simulink model "DroneModelSimulink"  (R2024b)
settings: Solver=VariableStepAuto  StartTime=0.0  StopTime=10  RelTol=1e-3
libraries: slpidlib x3, simulink x1
settings Model: Creator=ewert  LastModifiedBy=asus
settings SolverCC: AlgebraicLoopSolver=TrustRegion
settings DataIOCC: ReturnWorkspaceOutputs=off
settings DebuggingCC: UnconnectedInputMsg=warning  UnconnectedOutputMsg=warning  UnconnectedLineMsg=warning  ArithmeticOperatorsInVariantConditions=warning
settings ModelReferenceCC: EnableRefExpFcnMdlSchedulingChecks=on
settings SFSimCC: SimUseLocalCustomCode=off  CustomCodeUndefinedFunction=UseInterfaceOnly
settings RTWCC: RTWUseLocalCustomCode=off  GPUComputeCapability=3.5
settings CodeAppCC: StateflowObjectComments=on

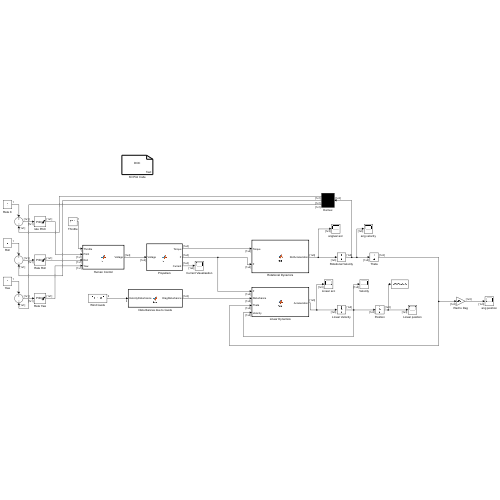
[thumbnail: Simulink's stored preview of the top-level diagram]
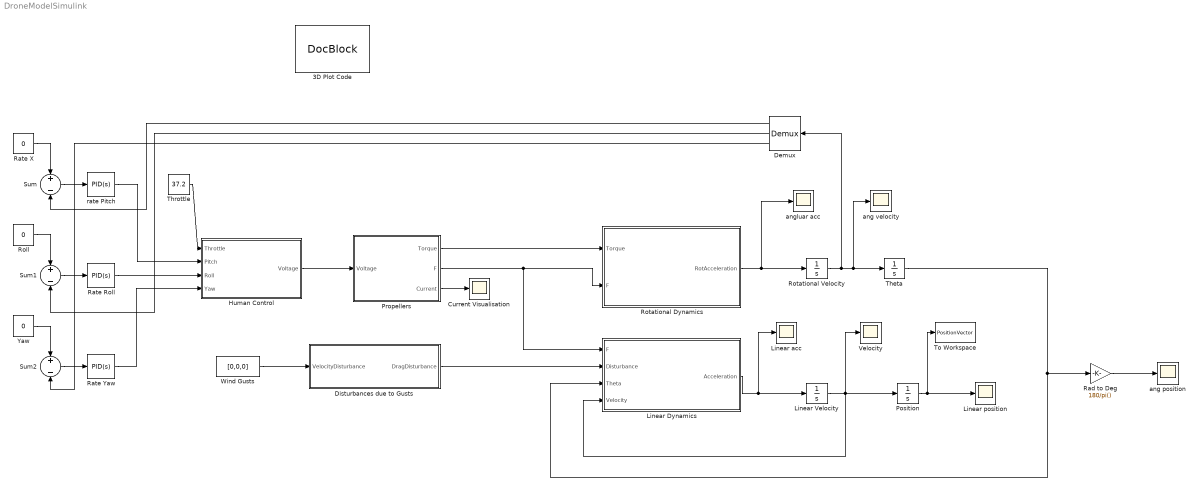
== system DroneModelSimulink ==
  3D Plot Code : simulink/Model-Wide Utilities/DocBlock  DocumentType=Text
      content=|
      | % Use this sample code once the simulation is completed to export 3D plot and visualize the drone's behavior
      | %----------------------------------
      | data3D = squeeze(PositionVector);
      | X = data3D(1, :);
      | Y = data3D(2, :);
      | Z = data3D(3, :);
      | figure;
      | plot3(X, Y, Z, '-r');
      | grid on;
      | xlabel('X');
      | ylabel('Y');
      | zlabel('Z');
      | title('3D Plot from Pos Data');
      | %----------------------------------
  "Current Visualisation " : Scope
  Demux : Demux  Outputs=3
  Disturbances due to Gusts : MATLAB Function  TreatAsAtomicUnit=on
  Human Control : MATLAB Function  TreatAsAtomicUnit=on
  Linear Dynamics : MATLAB Function  TreatAsAtomicUnit=on
  Linear Velocity : Integrator
  Linear acc : Scope
  Linear position : Scope
  Position : Integrator
  Propellers : MATLAB Function  TreatAsAtomicUnit=on
  Rad to Deg : Gain  Gain=180/pi()
  Rate Roll : slpidlib/PID Controller  Controller=PID  Form=Parallel  TimeDomain=Continuous-time  UseExternalTs=off  SampleTime=-1  IntegratorMethod=Forward Euler  FilterMethod=Forward Euler  ControllerParametersSource=internal  P=10  I=5  UseKiTs=off  D=0  UseExternalDerivativeSource=off  N=100  UseFilter=on  TunerSelectOption=Transfer Function Based (PID Tuner App)  InitialConditionSource=internal  InitialConditionForIntegrator=0  InitialConditionForFilter=0  DifferentiatorICPrevScaledInput=0  ExternalReset=none  TrackingMode=off  Kt=1  LimitOutput=on  SatLimitsSource=internal  UpperSaturationLimit=100  LowerSaturationLimit=0  LinearizeAsGain=on  AntiWindupMode=clamping  Kb=1  LimitIntegrator=off  UpperIntegratorSaturationLimit=inf  LowerIntegratorSaturationLimit=-inf  POutMin=[]  POutMax=[]  IOutMin=[]  IOutMax=[]  DOutMin=[]  DOutMax=[]  NOutMin=[]  NOutMax=[]  SumOutMin=[]  SumOutMax=[]  SaturationOutMin=[]  SaturationOutMax=[]  PParamMin=[]  PParamMax=[]  IParamMin=[]  IParamMax=[]  DParamMin=[]  DParamMax=[]  NParamMin=[]  NParamMax=[]  KbParamMin=[]  KbParamMax=[]  KtParamMin=[]  KtParamMax=[]  KbOutMin=[]  KbOutMax=[]  KtOutMin=[]  KtOutMax=[]  IntegratorOutMin=[]  IntegratorOutMax=[]  FilterOutMin=[]  FilterOutMax=[]  SumI1OutMin=[]  SumI1OutMax=[]  SumI2OutMin=[]  SumI2OutMax=[]  SumI3OutMin=[]  SumI3OutMax=[]  SumI4OutMin=[]  SumI4OutMax=[]  SumDOutMin=[]  SumDOutMax=[]  DifferentiatorOutMin=[]  DifferentiatorOutMax=[]  FilterDiffOutCoefMin=[]  FilterDiffOutCoefMax=[]  ReciprocalOutMin=[]  ReciprocalOutMax=[]  SumDenOutMin=[]  SumDenOutMax=[]  SumNumOutMin=[]  SumNumOutMax=[]  DivideOutMin=[]  DivideOutMax=[]  UdiffTsProdOutMin=[]  UdiffTsProdOutMax=[]  NTsProdOutMin=[]  NTsProdOutMax=[]  UintegralTsProdOutMin=[]  UintegralTsProdOutMax=[]  UngainTsProdOutMin=[]  UngainTsProdOutMax=[]  ClampingZeroOutDataTypeStr=Inherit: Inherit via back propagation  ClampingZeroOutMin=[]  ClampingZeroOutMax=[]  FilterDenConstantOutDataTypeStr=Inherit: Inherit via back propagation  FilterDenConstantOutMin=[]  FilterDenConstantOutMax=[]  PCopyOutDataTypeStr=Inherit: Inherit via back propagation  PCopyOutMin=[]  PCopyOutMax=[]  NCopyOutDataTypeStr=Inherit: Inherit via back propagation  NCopyOutMin=[]  NCopyOutMax=[]  IntegratorContinuousStateAttributes=''  IntegratorStateMustResolveToSignalObject=off  IntegratorRTWStateStorageClass=Auto  FilterContinuousStateAttributes=''  FilterStateMustResolveToSignalObject=off  FilterRTWStateStorageClass=Auto  ParallelPVariant=InternalParameters  IdealPVariant=Disabled  IVariant=InternalParameters  DVariant=InternalParameters  IntegratorVariant=Continuous  SatVariant=Enabled  AWVariant=ContClampingParallel  PCopyVariant=Disabled  TRVariant=Disabled  FdbkBlocksVariant=Forward  IdealPFdbkVariant=Disabled  SatFdbkVariant=Disabled  DerivativeFilterVariant=ContFilter  NVariant=InternalParameters  NCopyVariant=Disabled  FilterICVariant=InternalICsFilter  IntegratorICVariant=InternalICs  ExternalResetVariant=Disabled  TRSumVariant=Passthrough  SumFdbkVariant=Disabled  SumVariant=Sum_PID  TsampFilterVariant=InternalTs  TsampNgainVariant=Passthrough  TsampIntegralVariant=Disabled_SignalSpec  ExternalSaturationOutDataTypeStr=Inherit: Same as second input  DerivativeSourceVariant=ErrorSignal  PreIntVariant=InternalPreInt
  Rate X : Constant  Value=0
  Rate Yaw : slpidlib/PID Controller  Controller=PID  Form=Parallel  TimeDomain=Continuous-time  UseExternalTs=off  SampleTime=-1  IntegratorMethod=Forward Euler  FilterMethod=Forward Euler  ControllerParametersSource=internal  P=5  I=0.5  UseKiTs=off  D=0  UseExternalDerivativeSource=off  N=100  UseFilter=on  TunerSelectOption=Transfer Function Based (PID Tuner App)  InitialConditionSource=internal  InitialConditionForIntegrator=0  InitialConditionForFilter=0  DifferentiatorICPrevScaledInput=0  ExternalReset=none  TrackingMode=off  Kt=1  LimitOutput=on  SatLimitsSource=internal  UpperSaturationLimit=100  LowerSaturationLimit=0  LinearizeAsGain=on  AntiWindupMode=clamping  Kb=1  LimitIntegrator=off  UpperIntegratorSaturationLimit=inf  LowerIntegratorSaturationLimit=-inf  POutMin=[]  POutMax=[]  IOutMin=[]  IOutMax=[]  DOutMin=[]  DOutMax=[]  NOutMin=[]  NOutMax=[]  SumOutMin=[]  SumOutMax=[]  SaturationOutMin=[]  SaturationOutMax=[]  PParamMin=[]  PParamMax=[]  IParamMin=[]  IParamMax=[]  DParamMin=[]  DParamMax=[]  NParamMin=[]  NParamMax=[]  KbParamMin=[]  KbParamMax=[]  KtParamMin=[]  KtParamMax=[]  KbOutMin=[]  KbOutMax=[]  KtOutMin=[]  KtOutMax=[]  IntegratorOutMin=[]  IntegratorOutMax=[]  FilterOutMin=[]  FilterOutMax=[]  SumI1OutMin=[]  SumI1OutMax=[]  SumI2OutMin=[]  SumI2OutMax=[]  SumI3OutMin=[]  SumI3OutMax=[]  SumI4OutMin=[]  SumI4OutMax=[]  SumDOutMin=[]  SumDOutMax=[]  DifferentiatorOutMin=[]  DifferentiatorOutMax=[]  FilterDiffOutCoefMin=[]  FilterDiffOutCoefMax=[]  ReciprocalOutMin=[]  ReciprocalOutMax=[]  SumDenOutMin=[]  SumDenOutMax=[]  SumNumOutMin=[]  SumNumOutMax=[]  DivideOutMin=[]  DivideOutMax=[]  UdiffTsProdOutMin=[]  UdiffTsProdOutMax=[]  NTsProdOutMin=[]  NTsProdOutMax=[]  UintegralTsProdOutMin=[]  UintegralTsProdOutMax=[]  UngainTsProdOutMin=[]  UngainTsProdOutMax=[]  ClampingZeroOutDataTypeStr=Inherit: Inherit via back propagation  ClampingZeroOutMin=[]  ClampingZeroOutMax=[]  FilterDenConstantOutDataTypeStr=Inherit: Inherit via back propagation  FilterDenConstantOutMin=[]  FilterDenConstantOutMax=[]  PCopyOutDataTypeStr=Inherit: Inherit via back propagation  PCopyOutMin=[]  PCopyOutMax=[]  NCopyOutDataTypeStr=Inherit: Inherit via back propagation  NCopyOutMin=[]  NCopyOutMax=[]  IntegratorContinuousStateAttributes=''  IntegratorStateMustResolveToSignalObject=off  IntegratorRTWStateStorageClass=Auto  FilterContinuousStateAttributes=''  FilterStateMustResolveToSignalObject=off  FilterRTWStateStorageClass=Auto  ParallelPVariant=InternalParameters  IdealPVariant=Disabled  IVariant=InternalParameters  DVariant=InternalParameters  IntegratorVariant=Continuous  SatVariant=Enabled  AWVariant=ContClampingParallel  PCopyVariant=Disabled  TRVariant=Disabled  FdbkBlocksVariant=Forward  IdealPFdbkVariant=Disabled  SatFdbkVariant=Disabled  DerivativeFilterVariant=ContFilter  NVariant=InternalParameters  NCopyVariant=Disabled  FilterICVariant=InternalICsFilter  IntegratorICVariant=InternalICs  ExternalResetVariant=Disabled  TRSumVariant=Passthrough  SumFdbkVariant=Disabled  SumVariant=Sum_PID  TsampFilterVariant=InternalTs  TsampNgainVariant=Passthrough  TsampIntegralVariant=Disabled_SignalSpec  ExternalSaturationOutDataTypeStr=Inherit: Same as second input  DerivativeSourceVariant=ErrorSignal  PreIntVariant=InternalPreInt
  Roll : Constant  Value=0
  Rotational Dynamics : MATLAB Function  TreatAsAtomicUnit=on
  Rotational Velocity : Integrator
  Sum : Sum  Inputs=+-
  Sum1 : Sum  Inputs=+-
  Sum2 : Sum  Inputs=+-
  Theta : Integrator
  Throttle : Constant  Value=37.2
  To Workspace : ToWorkspace  VariableName=PositionVector  SampleTime=-1
      settings: Save2DSignal=2-D array (concatenate along first dimension)
  "Velocity " : Scope
  Wind Gusts : Constant  Value=[0,0,0]
  Yaw : Constant  Value=0
  ang position : Scope
  ang velocity : Scope
  angluar acc : Scope
  rate Pitch : slpidlib/PID Controller  Controller=PID  Form=Parallel  TimeDomain=Continuous-time  UseExternalTs=off  SampleTime=-1  IntegratorMethod=Forward Euler  FilterMethod=Forward Euler  ControllerParametersSource=internal  P=10  I=5  UseKiTs=off  D=0  UseExternalDerivativeSource=off  N=100  UseFilter=on  TunerSelectOption=Transfer Function Based (PID Tuner App)  InitialConditionSource=internal  InitialConditionForIntegrator=0  InitialConditionForFilter=0  DifferentiatorICPrevScaledInput=0  ExternalReset=none  TrackingMode=off  Kt=1  LimitOutput=on  SatLimitsSource=internal  UpperSaturationLimit=100  LowerSaturationLimit=0  LinearizeAsGain=on  AntiWindupMode=clamping  Kb=1  LimitIntegrator=off  UpperIntegratorSaturationLimit=inf  LowerIntegratorSaturationLimit=-inf  POutMin=[]  POutMax=[]  IOutMin=[]  IOutMax=[]  DOutMin=[]  DOutMax=[]  NOutMin=[]  NOutMax=[]  SumOutMin=[]  SumOutMax=[]  SaturationOutMin=[]  SaturationOutMax=[]  PParamMin=[]  PParamMax=[]  IParamMin=[]  IParamMax=[]  DParamMin=[]  DParamMax=[]  NParamMin=[]  NParamMax=[]  KbParamMin=[]  KbParamMax=[]  KtParamMin=[]  KtParamMax=[]  KbOutMin=[]  KbOutMax=[]  KtOutMin=[]  KtOutMax=[]  IntegratorOutMin=[]  IntegratorOutMax=[]  FilterOutMin=[]  FilterOutMax=[]  SumI1OutMin=[]  SumI1OutMax=[]  SumI2OutMin=[]  SumI2OutMax=[]  SumI3OutMin=[]  SumI3OutMax=[]  SumI4OutMin=[]  SumI4OutMax=[]  SumDOutMin=[]  SumDOutMax=[]  DifferentiatorOutMin=[]  DifferentiatorOutMax=[]  FilterDiffOutCoefMin=[]  FilterDiffOutCoefMax=[]  ReciprocalOutMin=[]  ReciprocalOutMax=[]  SumDenOutMin=[]  SumDenOutMax=[]  SumNumOutMin=[]  SumNumOutMax=[]  DivideOutMin=[]  DivideOutMax=[]  UdiffTsProdOutMin=[]  UdiffTsProdOutMax=[]  NTsProdOutMin=[]  NTsProdOutMax=[]  UintegralTsProdOutMin=[]  UintegralTsProdOutMax=[]  UngainTsProdOutMin=[]  UngainTsProdOutMax=[]  ClampingZeroOutDataTypeStr=Inherit: Inherit via back propagation  ClampingZeroOutMin=[]  ClampingZeroOutMax=[]  FilterDenConstantOutDataTypeStr=Inherit: Inherit via back propagation  FilterDenConstantOutMin=[]  FilterDenConstantOutMax=[]  PCopyOutDataTypeStr=Inherit: Inherit via back propagation  PCopyOutMin=[]  PCopyOutMax=[]  NCopyOutDataTypeStr=Inherit: Inherit via back propagation  NCopyOutMin=[]  NCopyOutMax=[]  IntegratorContinuousStateAttributes=''  IntegratorStateMustResolveToSignalObject=off  IntegratorRTWStateStorageClass=Auto  FilterContinuousStateAttributes=''  FilterStateMustResolveToSignalObject=off  FilterRTWStateStorageClass=Auto  ParallelPVariant=InternalParameters  IdealPVariant=Disabled  IVariant=InternalParameters  DVariant=InternalParameters  IntegratorVariant=Continuous  SatVariant=Enabled  AWVariant=ContClampingParallel  PCopyVariant=Disabled  TRVariant=Disabled  FdbkBlocksVariant=Forward  IdealPFdbkVariant=Disabled  SatFdbkVariant=Disabled  DerivativeFilterVariant=ContFilter  NVariant=InternalParameters  NCopyVariant=Disabled  FilterICVariant=InternalICsFilter  IntegratorICVariant=InternalICs  ExternalResetVariant=Disabled  TRSumVariant=Passthrough  SumFdbkVariant=Disabled  SumVariant=Sum_PID  TsampFilterVariant=InternalTs  TsampNgainVariant=Passthrough  TsampIntegralVariant=Disabled_SignalSpec  ExternalSaturationOutDataTypeStr=Inherit: Same as second input  DerivativeSourceVariant=ErrorSignal  PreIntVariant=InternalPreInt
  wires:
  Propellers/1(Torque) -> Rotational Dynamics/1(Torque)
  Propellers/2(F) -> Linear Dynamics/1(F), Rotational Dynamics/2(F)
  Rotational Dynamics/1(RotAcceleration) -> angluar acc/1, Rotational Velocity/1
  Rotational Velocity/1 -> Demux/1, ang velocity/1, Theta/1
  Theta/1 -> Rad to Deg/1, Linear Dynamics/3(Theta)
  Linear Dynamics/1(Acceleration) -> Linear acc/1, Linear Velocity/1
  Linear Velocity/1 -> "Velocity "/1, Position/1, Linear Dynamics/4(Velocity)
  Disturbances due to Gusts/1(DragDisturbance) -> Linear Dynamics/2(Disturbance)
  Wind Gusts/1 -> Disturbances due to Gusts/1(VelocityDisturbance)
  Human Control/1(Voltage) -> Propellers/1(Voltage)
  Rad to Deg/1 -> ang position/1
  Propellers/3(Current) -> "Current Visualisation "/1
  Rate X/1 -> Sum/1
  Sum/1 -> rate Pitch/1
  Demux/1 -> Sum/2
  rate Pitch/1 -> Human Control/2(Pitch)
  Throttle/1 -> Human Control/1(Throttle)
  Rate Roll/1 -> Human Control/3(Roll)
  Roll/1 -> Sum1/1
  Sum1/1 -> Rate Roll/1
  Demux/2 -> Sum1/2
  Rate Yaw/1 -> Human Control/4(Yaw)
  Yaw/1 -> Sum2/1
  Sum2/1 -> Rate Yaw/1
  Demux/3 -> Sum2/2
  Position/1 -> To Workspace/1, Linear position/1

== matlab function DroneModelSimulink/Rotational Dynamics ==
  data: Torque input; RotAcceleration output; F input
function RotAcceleration = fcn(Torque, F)
Moment=[0 0 0];
RotAcceleration=[0 0 0];
I=[0.003,0.003,0.007];
Moment(1)=(F(3)+F(4))*0.237/2-(F(1)+F(2))*0.237/2;
Moment(2)=(F(3)+F(2))*0.237/2-(F(1)+F(4))*0.237/2;
Moment(3)=Torque(4)-Torque(1)+Torque(2)-Torque(3);
for i=1:3
    RotAcceleration(i)=Moment(i)/I(i);
end

== matlab function DroneModelSimulink/Propellers ==
  data: Voltage input; Torque output; F output; Current output
function [Torque, F, Current] = fcn(Voltage)
RPM=[0 0 0 0];
F=[0 0 0 0];
Current=[0 0 0 0];
Torque=[0 0 0 0];
for i=1:4
    RPM(i) = -2.6931 * Voltage(i)^3 + 1400 * Voltage(i);
    Ct = 2 * 10^-15 * RPM(i)^3 - 4 * 10^-11 * RPM(i)^2 + 3 * 10^-7 * RPM(i) + 0.1013;
    F(i) = Ct * 1.225 * (RPM(i)/60)^2 * 0.2^4;
    Torque(i) = 4 * 10^-14 * RPM(i)^3 + 8 * 10^-12 * RPM(i)^2 + 3 * 10^-6 * RPM(i);
    Current(i) = 1400 *  Torque(i);
end

== matlab function DroneModelSimulink/Linear Dynamics ==
  data: F input; Acceleration output; Disturbance input; Theta input; Velocity input
function Acceleration  = fcn(F,Disturbance,Theta,Velocity)
m=0.743;
g=9.81;
A=[0.0197 0.0197 0.0512];
rho=1.225;
Cd=1;

Acceleration=[0 0 0];
Force=[0 0 0];
Fprop=[0;0;0];

Fprop(1,1)=sin(Theta(2))*cos(Theta(1))*(F(1)+F(2)+F(3)+F(4));
Fprop(2,1)=sin(Theta(1))*cos(Theta(2))*(F(1)+F(2)+F(3)+F(4));

Fprop(3,1)=(F(1)+F(2)+F(3)+F(4))*cos(Theta(1))*cos(Theta(2));

ThetaXY=-atan2(Fprop(1),Fprop(2));
XY2D=sqrt(Fprop(1)^2+Fprop(2)^2);
if Fprop(3)>=0
    Fprop(1)=XY2D*sin(Theta(3)+ThetaXY);
    Fprop(2)=XY2D*cos(Theta(3)+ThetaXY);
else
     Fprop(1)=XY2D*sin(-Theta(3)+ThetaXY);
    Fprop(2)=XY2D*cos(-Theta(3)+ThetaXY);
end
    
if Velocity(1)<0
Force(1)=Fprop(1)-Disturbance(1)+0.5*rho*Velocity(1)^2*A(1)*Cd;
else 
    Force(1)=Fprop(1)-Disturbance(1)-0.5*rho*Velocity(1)^2*A(1)*Cd;
end

if Velocity(2)<0
Force(2)=Fprop(2)-Disturbance(2)+0.5*rho*Velocity(2)^2*A(2)*Cd;
else 
    Force(2)=Fprop(2)-Disturbance(2)-0.5*rho*Velocity(2)^2*A(2)*Cd;
end

if Velocity(3)<0
Force(3)=Fprop(3)+0.5*rho*Velocity(3)^2*A(3)*Cd-m*g-Disturbance(3);
else 
Force(3)=Fprop(3)-0.5*rho*Velocity(3)^2*A(3)*Cd-m*g-Disturbance(3);
end

for i=1:3
    Acceleration(i)=Force(i)/m;
end

== matlab function DroneModelSimulink/Disturbances due to Gusts ==
  data: VelocityDisturbance input; DragDisturbance output
function DragDisturbance = fcn(VelocityDisturbance)
A=[0.0197 0.0197 0.0197*2*1.3];
DragDisturbance=[0 0 0];
rho=1.225;
Cd=1;

for i=1:3
    if VelocityDisturbance(i)<0
        DragDisturbance(i)=-0.5*rho*VelocityDisturbance(i)^2*A(i)*Cd;
    else
        DragDisturbance(i)=0.5*rho*VelocityDisturbance(i)^2*A(i)*Cd;
    end
end

== matlab function DroneModelSimulink/Human Control ==
  data: Throttle input; Voltage output; Pitch input; Roll input; Yaw input
function Voltage = fcn(Throttle, Pitch, Roll, Yaw)
Correct=0;
if (Pitch/2+Roll/2+Yaw/2)>(100-Throttle)
    Correct=((Pitch/2+Roll/2+Yaw/2)-(100-Throttle));
end
if (Pitch/2+Roll/2+Yaw/2)>(Throttle)
    if Correct<((Pitch/2+Roll/2+Yaw/2)-(Throttle))
       Correct=((Pitch/2+Roll/2+Yaw/2)-(Throttle));
    end
end
%factors on correct to be relevant to the comparisons above which look at
%the actual application.
if Correct~=0
Pitch=Pitch-Correct/3*2;
Roll=Roll-Correct/3*2;
Yaw=Yaw-Correct/3*2;
end

Voltage=[(Throttle-Pitch/2-Roll/2-Yaw/2)*11.4/100 (Throttle-Pitch/2+Roll/2+Yaw/2)*11.4/100 (Throttle+Pitch/2+Roll/2-Yaw/2)*11.4/100 (Throttle+Pitch/2-Roll/2+Yaw/2)*11.4/100];
